simulink model "Lab8_p2_Proportional_13b"  (R2013b)
settings: Solver=FixedStepDiscrete  SolverMode=SingleTasking  StartTime=0.0  StopTime=inf  FixedStep=sim_step_size  RelTol=1e-3
PreLoadFcn:
  | % Default parameters
  | C2D = 0.5;
  | Vs = 4.5;
  | %
  | sim_step_size = 0.03;
  | Kp = 0.1
settings Model: SimulationMode=external  ExtModeTrigDuration=2  Creator=nding  LastModifiedBy=nding
settings OptimizationCC: OptimizeModelRefInitCode=on  LifeSpan=1
settings DebuggingCC: SolverPrmCheckMsg=none
settings HardwareCC: ProdBitPerInt=16  ProdBitPerPointer=8  ProdIntDivRoundTo=Zero  ProdEndianess=LittleEndian  ProdWordSize=8  ProdHWDeviceType=Atmel->AVR
settings RTWCC: SystemTargetFile=realtime.tlc  GenerateMakefile=off  TemplateMakefile=realtime.tmf  Description=Run on Target Hardware  RTWVerbose=off  ProcessScript=realtime_make_rtw_hook
settings STFCustomTargetCC: TargetLibSuffix=.a  GenerateSampleERTMain=on  ERTCustomFileBanners=on  SupportNonInlinedSFcns=off  SupportVariableSizeSignals=on  MATLABClassNameForMDSCustomization=Simulink.SoftwareTarget.ERTCustomization  GRTInterface=off  SystemTargetFile=realtime.tlc
settings ERTTargetCC: CodeReplacementLibrary=ANSI_C  GenerateSampleERTMain=on  ParMdlRefBuildCompliant=off  CompOptLevelCompliant=off  ConcurrentExecutionCompliant=off  CombineOutputUpdateFcns=off  ERTFirstTimeCompliant=off  SupportContinuousTime=on  SupportVariableSizeSignals=on  ModelStepFunctionPrototypeControlCompliant=off  CPPClassGenCompliant=off  ExtMode=on  ExtModeTransport=3  ExtModeMexArgs=0 11 115200 30  InlinedParameterPlacement=NonHierarchical  ERTSrcFileBannerTemplate=realtime_code_template.cgt  ERTHdrFileBannerTemplate=realtime_code_template.cgt  ERTDataSrcFileTemplate=realtime_code_template.cgt  ERTDataHdrFileTemplate=realtime_code_template.cgt  ERTCustomFileTemplate=realtime_file_process.tlc

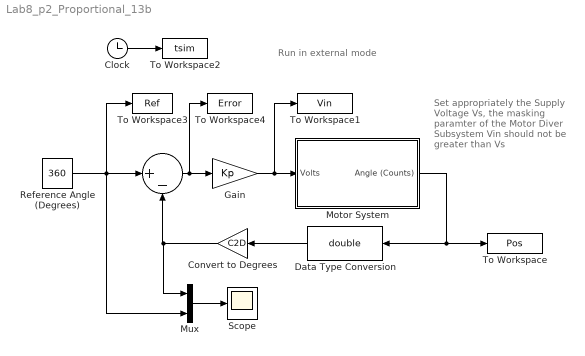
== system Lab8_p2_Proportional_13b ==
  note: Set appropriately the Supply
      | Voltage Vs, the masking paramter
      | of the Motor Diver Subsystem
      |
      | Vin should not  be greater than Vs
  note: Run in external mode
  " " : Sum  Inputs=|+-
  Clock : Clock
  Convert to Degrees : Gain  Gain=C2D
  Data Type Conversion : DataTypeConversion  OutDataTypeStr=double
  Gain : Gain  Gain=Kp
  Motor System : Subsystem
  Mux : Mux  Inputs=2
  Reference Angle (Degrees) : Constant  Value=360
  Scope : Scope
      settings: YMin=290  YMax=400
  To Workspace : ToWorkspace  VariableName=Pos  SampleTime=-1
  To Workspace1 : ToWorkspace  VariableName=Vin  SampleTime=-1
  To Workspace2 : ToWorkspace  VariableName=tsim  SampleTime=sim_step_size
  To Workspace3 : ToWorkspace  VariableName=Ref  SampleTime=-1
  To Workspace4 : ToWorkspace  VariableName=Error  SampleTime=-1
  wires:
  Motor System/1(Angle (Counts)) -> To Workspace/1, Data Type Conversion/1
  Gain/1 -> To Workspace1/1, Motor System/1(Volts)
  Clock/1 -> To Workspace2/1
  " "/1 -> To Workspace4/1, Gain/1
  Reference Angle (Degrees)/1 -> To Workspace3/1, " "/1, Mux/2
  Data Type Conversion/1 -> Convert to Degrees/1
  Convert to Degrees/1 -> Mux/1, " "/2
  Mux/1 -> Scope/1

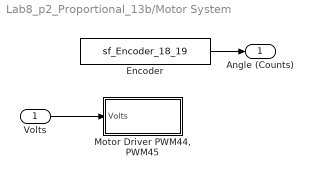
== system Lab8_p2_Proportional_13b/Motor System ==
  Volts : Inport
  Encoder : S-Function  InitFcn=try, set_param(gcb,'FunctionName','sf_Encoder_18_19'), end  FunctionName=sf_Encoder_18_19  Parameters=uint8(0),uint8(18),uint8(19)  SFunctionModules=sf_Encoder_18_19_wrapper  EnableBusSupport=off  mask(S-Function Builder){}
      mask init:
      | val = [[.9  0.75 0.75 1 1 .9 .9 1]',[1 1 0.75 0.75 .9 .9 1 .9]'];try , sys = get_param(gcb,'SfunBuilderFcnName');if isempty(sys), sys = get_param(gcb,'FunctionName'); end,catch, sys = get_param(gcb,'FunctionName'); end
      settings: CopyFcn=set_param(gcbh,'LinkStatus','none')  PreSaveFcn=try, set_param(gcb,'FunctionName','sf_Encoder_18_19'), end  OpenFcn=sfunctionwizard(gcbh)
      mask Display: plot(val(:,1),val(:,2)),disp(sys), port_label('output',1,'pos')
  "Motor Driver PWM44, PWM45" : Subsystem  mask{Vs=Vs, Delta=0}
      mask prompts: Vs "Supply Voltage Vs: USB 4.5v; Battery 9v"; Delta "PWM Offset Delta: 0-255"
      mask init:
      | Vusb=4.5;
      | Vbat=9.0;
      mask DialogControl T Prompt: Specify Motor Supply Voltage and PWM Offset
  Angle (Counts) : Outport
  wires:
  Encoder/1 -> Angle (Counts)/1
  Volts/1 -> "Motor Driver PWM44, PWM45"/1(Volts)

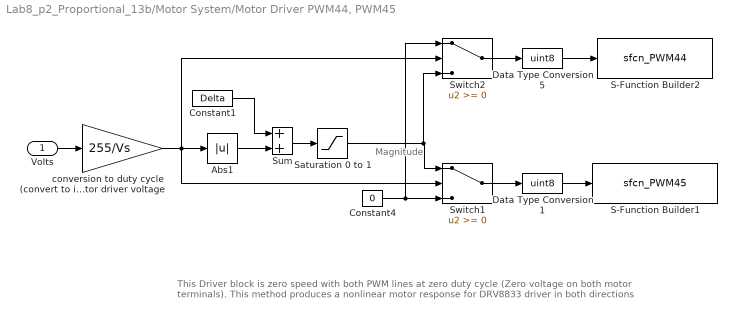
== system Lab8_p2_Proportional_13b/Motor System/Motor Driver PWM44, PWM45 ==
  note: Magnitude
  note: This Driver block is zero speed with both PWM lines at zero duty cycle  (Zero voltage on both motor terminals).
      | This method produces a nonlinear motor response for DRV8833 driver in both directions
  Volts : Inport
  Abs1 : Abs
  Constant1 : Constant  Value=Delta
  Constant4 : Constant  Value=0
  Data Type Conversion1 : DataTypeConversion  OutDataTypeStr=uint8
  Data Type Conversion5 : DataTypeConversion  OutDataTypeStr=uint8
  S-Function Builder1 : S-Function  InitFcn=try, set_param(gcb,'FunctionName','sfcn_PWM45'), end  FunctionName=sfcn_PWM45  Parameters=uint8(45)  SFunctionModules=sfcn_PWM45_wrapper  EnableBusSupport=off  mask(S-Function Builder){}
      mask init: same as Lab8_p2_Proportional_13b/Motor System/Encoder
      settings: CopyFcn=set_param(gcbh,'LinkStatus','none')  PreSaveFcn=try, set_param(gcb,'FunctionName','sfcn_PWM45'), end  OpenFcn=sfunctionwizard(gcbh)
      mask Display: plot(val(:,1),val(:,2)),disp(sys), port_label('input',1,'in')
  S-Function Builder2 : S-Function  InitFcn=try, set_param(gcb,'FunctionName','sfcn_PWM44'), end  FunctionName=sfcn_PWM44  Parameters=uint8(44)  SFunctionModules=sfcn_PWM44_wrapper  EnableBusSupport=off  mask(S-Function Builder){}
      mask init: same as Lab8_p2_Proportional_13b/Motor System/Encoder
      settings: CopyFcn=set_param(gcbh,'LinkStatus','none')  PreSaveFcn=try, set_param(gcb,'FunctionName','sfcn_PWM44'), end  OpenFcn=sfunctionwizard(gcbh)
      mask Display: plot(val(:,1),val(:,2)),disp(sys), port_label('input',1,'in')
  Saturation 0 to 1 : Saturate  UpperLimit=255  LowerLimit=0
  Sum : Sum
  Switch1 : Switch
  Switch2 : Switch
  conversion to duty cycle (convert to int) denominator is motor driver voltage : Gain  Gain=255/Vs  OutDataTypeStr=int16
  wires:
  Constant1/1 -> Sum/1
  Sum/1 -> Saturation 0 to 1/1
  Abs1/1 -> Sum/2
  Data Type Conversion1/1 -> S-Function Builder1/1
  Data Type Conversion5/1 -> S-Function Builder2/1
  Switch1/1 -> Data Type Conversion1/1
  Switch2/1 -> Data Type Conversion5/1
  Saturation 0 to 1/1 -> Switch1/1, Switch2/3
  Constant4/1 -> Switch1/3, Switch2/1
  conversion to duty cycle (convert to int) denominator is motor driver voltage/1 -> Switch2/2, Abs1/1, Switch1/2
  Volts/1 -> conversion to duty cycle (convert to int) denominator is motor driver voltage/1
